simulink model "CochlearImplant_SIL"  (R2026b)
settings: Solver=FixedStepDiscrete  StopTime=5
PreLoadFcn:
  | addpath(fileparts(which('CochlearImplant_SIL')));
PostLoadFcn:
  | load speech_dft.mat
InitFcn:
  | dspcochlearfilterdesign;
  | source_type = 2;% 2 = Speech signal (1=Chirp)
  | filter_type = 1;% 1 = Cascade multirate FIR
  | noise_type  = 0;% 0 = no noise
  | denoise     = 0;% 0 = denoise off
StopFcn:
  | % Refresh OrigSignal/SynSignal in base from the latest run so the
  | % Play buttons never use stale data (robust to Single-simulation-output).
  | try
  |     if evalin('base','exist(''logsout'',''var'')')
  |         ls = evalin('base','logsout');
  |         if isa(ls,'Simulink.SimulationData.Dataset')
  |             if any(strcmp(ls.getElementNames,'InputSignal'))
  |                 assignin('base','OrigSignal', ls.get('InputSignal').Values.Data(:));
  |             end
  |             if any(strcmp(ls.getElementNames,'ReconSignal'))
  |                 assignin('base','SynSignal', ls.get('ReconSignal').Values.Data(:));
  |             end
  |         end
  |     end
  | catch ME
  |     warning('CochlearDemo:StopFcn','Could not refresh audio vars: %s', ME.message);
  | end
values from neighbouring files (symbols this model uses):
  cochleardemo_bpf = dsp.FIRFilter('Numerator', firls(32,[0 .22 .42 .54 .74 1], [0 0 1 1 0 0]))    [dspcochlearfilterdesign.m]
  cochleardemo_fir_hi = dsp.FIRFilter('Numerator', firls(32,[0 .62 .82 1], [0 0 1 1]))    [dspcochlearfilterdesign.m]
  cochleardemo_fir_lo = dsp.FIRFilter('Numerator', firls(32,[0 .62 .82 1], [1 1 0 0]))    [dspcochlearfilterdesign.m]
  cochleardemo_hpf = dsp.FIRFilter('Numerator', firls(32,[0 .54 .74 1], [0 0 1 1]))    [dspcochlearfilterdesign.m]
  cochleardemo_lpf = dsp.FIRFilter('Numerator', firls(32,[0 .22 .42  1], [1 1 0 0]))    [dspcochlearfilterdesign.m]
  fs = evalin('base', 'fs')    [plotFilterBankResponses.m]    (also in speech_dft.mat = 22050)
undefined symbols (not defined in the file or in its folder): cochleardemo_inputFilter, dfilt
libraries: dsparch4 x16, dspmlti4 x3, dspsrcs4 x1
settings Model: SILPILModeSetting=veronly  SimulationMode=software-in-the-loop (sil)  Creator=nkotwal  LastModifiedBy=jcchun
settings DataIOCC: ExternalInput=in  LoadExternalInput=on  ReturnWorkspaceOutputs=off  SignalLogging=off
settings OptimizationCC: DefaultParameterBehavior=Inlined  DifferentSizesBufferReuse=on  EfficientTunableParamExpr=on  EnhancedBackFolding=on  OptimizationCustomize=off  OptimizeBlockOrder=speed  PassReuseOutputArgsAs=Individual arguments  RemoveInternalMemoryZeroInit=on  RemoveRootLevelIOMemoryZeroInit=on
settings DebuggingCC: ParameterTunabilityLossMsg=error
settings HardwareCC: ProdHWDeviceType=AMD->x86-64 (Linux 64)
settings SFSimCC: MATLABDynamicMemAlloc=off
settings RTWCC: DataTypeReplacement=CDataTypesFixedWidth  Description=Embedded Coder  GenCodeOnly=on  GenerateCodeMetricsReport=on  GenerateReport=on  GenerateTraceInfo=on  IncludeHyperlinkInReport=on  SystemTargetFile=ert.tlc  TemplateMakefile=ert_default_tmf
settings CodeAppCC: ForceParamTrailComments=on  IgnoreCustomStorageClasses=off  InsertBlockDesc=on  OperatorAnnotations=on  SFDataObjDesc=on  SimulinkDataObjDesc=on
settings ERTTargetCC: CombineSignalStateStructs=on  GenerateSampleERTMain=on  MaxIdInt16=INT16_MAX  MaxIdInt32=INT32_MAX  MaxIdInt64=INT64_MAX  MaxIdInt8=INT8_MAX  MaxIdUint16=UINT16_MAX  MaxIdUint32=UINT32_MAX  MaxIdUint64=UINT64_MAX  MaxIdUint8=UINT8_MAX  MinIdInt16=INT16_MIN  MinIdInt32=INT32_MIN  MinIdInt64=INT64_MIN  MinIdInt8=INT8_MIN

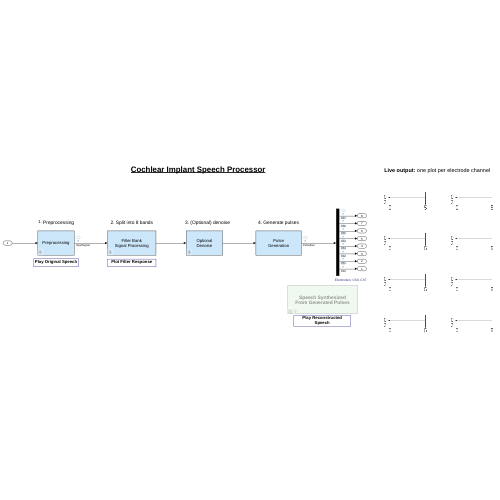
[thumbnail: Simulink's stored preview of the top-level diagram]
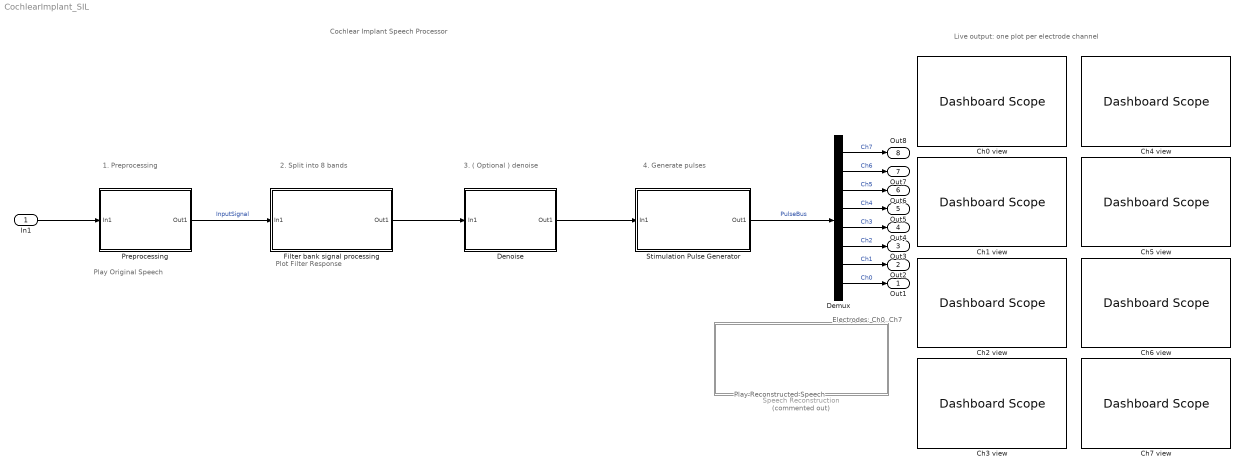
== system CochlearImplant_SIL ==
  note: Cochlear Implant Speech Processor
  note: 1. Preprocessing
  note: 2. Split into 8 bands
  note: 3. ( Optional ) denoise
  note: 4. Generate pulses
  note: Electrodes: Ch0..Ch7
  note: Live output: one plot per electrode channel
  note: Plot Filter Response
  note: Play Original Speech
  note: Play Reconstructed Speech
  In1 : Inport
  Ch0 view : DashboardScope  FontColor=[0.0, 0.0, 0.0]
  Ch1 view : DashboardScope  FontColor=[0.0, 0.0, 0.0]
  Ch2 view : DashboardScope  FontColor=[0.0, 0.0, 0.0]
  Ch3 view : DashboardScope  FontColor=[0.0, 0.0, 0.0]
  Ch4 view : DashboardScope  FontColor=[0.0, 0.0, 0.0]
  Ch5 view : DashboardScope  FontColor=[0.0, 0.0, 0.0]
  Ch6 view : DashboardScope  FontColor=[0.0, 0.0, 0.0]
  Ch7 view : DashboardScope  FontColor=[0.0, 0.0, 0.0]
  Demux : Demux  Outputs=8
  Denoise : Subsystem  mask{denoise=off}
      mask help: Apply soft thresholds to each filter bank output.
      mask Display: disp('Optional\nDenoise');
  Filter bank signal processing : Subsystem  mask(Filter bank signal processing){filter_type=Cascade multirate multi-stage FIR}
      mask prompts: filter_type "Filter bank:"
      mask help: Processes the input audio signal using a filter bank with eight subbands.
      mask TypeOptions filter_type: Cascade multirate multi-stage FIR | Parallel single-rate SOS IIR
      mask Display: disp('Filter Bank\nSignal Processing');
  Preprocessing : Subsystem  mask(Preprocessing){}
      mask Display: disp('Preprocessing');
  Speech Reconstruction : Subsystem  Commented=on  mask(Speech Synthesized From Generated Pulses){syn_mode=Play all channels at once}
      mask prompts: syn_mode "Synthesis mode:"
      mask help: Select whether to play all channels simultaneously or sequentially.
      mask TypeOptions syn_mode: Play all channels at once | Play channels sequentially
      mask Display: disp(sprintf('Speech Synthesized\nFrom Generated Pulses'));
  Stimulation Pulse Generator : Subsystem
      mask Display: disp('Pulse\nGeneration')
  Out1 : Outport
  Out2 : Outport  Port=2
  Out3 : Outport  Port=3
  Out4 : Outport  Port=4
  Out5 : Outport  Port=5
  Out6 : Outport  Port=6
  Out7 : Outport  Port=7
  Out8 : Outport  Port=8
  wires:
  Filter bank signal processing/1(Out1) -> Denoise/1(In1)
  Denoise/1(Out1) -> Stimulation Pulse Generator/1(In1)
  Stimulation Pulse Generator/1(Out1) -> Demux/1  "PulseBus"
  Preprocessing/1(Out1) -> Filter bank signal processing/1(In1)  "InputSignal"
  In1/1 -> Preprocessing/1(In1)
  Demux/8 -> Out1/1  "Ch0"
  Demux/7 -> Out2/1  "Ch1"
  Demux/6 -> Out3/1  "Ch2"
  Demux/5 -> Out4/1  "Ch3"
  Demux/4 -> Out5/1  "Ch4"
  Demux/3 -> Out6/1  "Ch5"
  Demux/2 -> Out7/1  "Ch6"
  Demux/1 -> Out8/1  "Ch7"

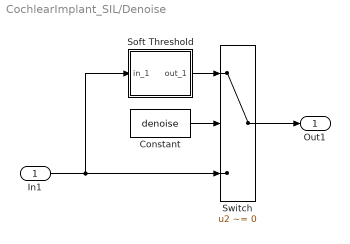
== system CochlearImplant_SIL/Denoise ==
  In1 : Inport
  Constant : Constant  Value=denoise
  Soft Threshold : Subsystem  mask(Soft Threshold){st=[0.5  0.3  0.2  0.2  0.2  0.2  0.2  0.2]}
      mask prompts: st "Vector of thresholds for each level:"
      mask help: Apply a soft threshold (deadzone transfer function) to each signal in the decomposition. First threshold applies to top-most filter bank output.
      mask init:
      | x=([-1 1 NaN 0 0 NaN -1 -.5 .5 1]+1)/2*.7+.15;
      | y=([0 0 NaN -1 1 NaN -1 0 0 1]+1)/2*.7+.05;
      mask Help: Vector of thresholds for each decomposition level.
      mask Display:
      | text(.1,.9,'Dead Zone')
      | plot(x,y)
  Switch : Switch  Criteria=u2 ~= 0  SaturateOnIntegerOverflow=off  InputSameDT=off
  Out1 : Outport  VectorParamsAs1DForOutWhenUnconnected=off
  wires:
  In1/1 -> Switch/3, Soft Threshold/1(in_1)
  Soft Threshold/1(out_1) -> Switch/1
  Switch/1 -> Out1/1
  Constant/1 -> Switch/2

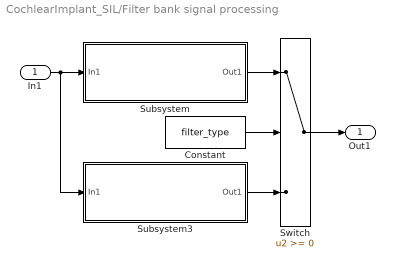
== system CochlearImplant_SIL/Filter bank signal processing ==
  In1 : Inport
  Constant : Constant  Value=filter_type
  Subsystem : Subsystem
      mask Display: disp('Cascade multirate multi-stage\nFIR filter bank');
  Subsystem3 : Subsystem
      mask Display: disp('Parallel single-rate\nSOS IIR filter bank');
  Switch : Switch  SaturateOnIntegerOverflow=off  InputSameDT=off
  Out1 : Outport  VectorParamsAs1DForOutWhenUnconnected=off
  wires:
  Switch/1 -> Out1/1
  In1/1 -> Subsystem3/1(In1), Subsystem/1(In1)
  Constant/1 -> Switch/2
  Subsystem3/1(Out1) -> Switch/3
  Subsystem/1(Out1) -> Switch/1

== system CochlearImplant_SIL/Preprocessing ==
  note: Input Preprocessing
  In1 : Inport
  Buffer : Buffer  N=8  ic=[0;0;0;0;0;3.0517578125e-05;-3.0517578125e-05;6.103515625e-05]
  DC Blocking Filter : DiscreteFilter  Numerator=cochleardemo_inputFilter.b  Denominator=cochleardemo_inputFilter.a  InputProcessing=Columns as channels (frame based)  FilterStructure=Direct form II transposed  a0EqualsOne=on  NumAccumDataTypeStr=Inherit: Same as product output  DenAccumDataTypeStr=Inherit: Same as product output
  stw : ToWorkspace  VariableName=OrigSignal  SampleTime=-1
      settings: Save2DSignal=2-D array (concatenate along first dimension)
  Out1 : Outport  VectorParamsAs1DForOutWhenUnconnected=off
  wires:
  DC Blocking Filter/1 -> Out1/1, stw/1
  Buffer/1 -> DC Blocking Filter/1
  In1/1 -> Buffer/1

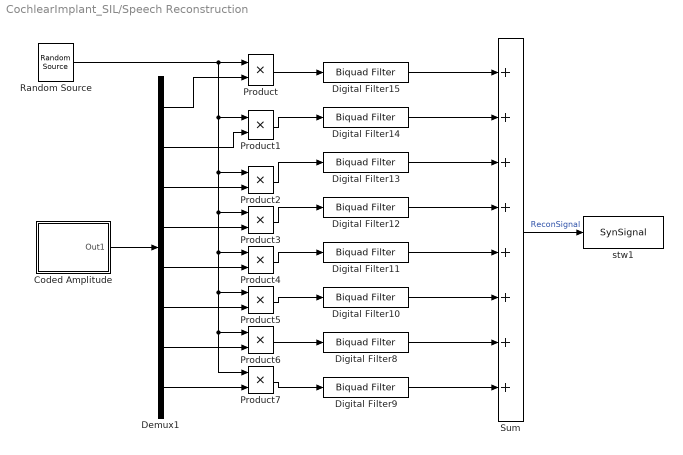
== system CochlearImplant_SIL/Speech Reconstruction ==
  Coded Amplitude : Subsystem
      mask Display: disp(['Speech' 10 'generated' 10 'pulses']);
  Demux1 : Demux  Outputs=8
  Digital Filter10 : dsparch4/Biquad Filter  FilterSource=Dialog parameters  CoeffSource=Specify via dialog  FilterObject=dfilt.df2tsos([1 0.3 0.4],[1 0.1 0.2])  IIRFiltStruct=Direct form II transposed  BiQuadCoeffs=cochleardemo_f2.sosMatrix  ScaleValues=cochleardemo_f2.ScaleValues  IC=0  ICnum=0  ICden=0  a0Flag=Error  optimizeScaleValues=on  ScaleValueMode=Specify via input port (g)  InputProcessing=Columns as channels (frame based)  roundingMode=Floor  overflowMode=off  scaleValueFracLength=14  denProdOutputFracLength=30  denAccumFracLength=30  secondMemoryFracLength=15
  Digital Filter11 : dsparch4/Biquad Filter  FilterSource=Dialog parameters  CoeffSource=Specify via dialog  FilterObject=dfilt.df2tsos([1 0.3 0.4],[1 0.1 0.2])  IIRFiltStruct=Direct form II transposed  BiQuadCoeffs=cochleardemo_f3.sosMatrix  ScaleValues=cochleardemo_f3.ScaleValues  IC=0  ICnum=0  ICden=0  a0Flag=Error  optimizeScaleValues=on  ScaleValueMode=Specify via input port (g)  InputProcessing=Columns as channels (frame based)  roundingMode=Floor  overflowMode=off  scaleValueFracLength=14  denProdOutputFracLength=30  denAccumFracLength=30  secondMemoryFracLength=15
  Digital Filter12 : dsparch4/Biquad Filter  FilterSource=Dialog parameters  CoeffSource=Specify via dialog  FilterObject=dfilt.df2tsos([1 0.3 0.4],[1 0.1 0.2])  IIRFiltStruct=Direct form II transposed  BiQuadCoeffs=cochleardemo_f4.sosMatrix  ScaleValues=cochleardemo_f4.ScaleValues  IC=0  ICnum=0  ICden=0  a0Flag=Error  optimizeScaleValues=on  ScaleValueMode=Specify via input port (g)  InputProcessing=Columns as channels (frame based)  roundingMode=Floor  overflowMode=off  scaleValueFracLength=14  denProdOutputFracLength=30  denAccumFracLength=30  secondMemoryFracLength=15
  Digital Filter13 : dsparch4/Biquad Filter  FilterSource=Dialog parameters  CoeffSource=Specify via dialog  FilterObject=dfilt.df2tsos([1 0.3 0.4],[1 0.1 0.2])  IIRFiltStruct=Direct form II transposed  BiQuadCoeffs=cochleardemo_f5.sosMatrix  ScaleValues=cochleardemo_f5.ScaleValues  IC=0  ICnum=0  ICden=0  a0Flag=Error  optimizeScaleValues=on  ScaleValueMode=Specify via input port (g)  InputProcessing=Columns as channels (frame based)  roundingMode=Floor  overflowMode=off  scaleValueFracLength=14  denProdOutputFracLength=30  denAccumFracLength=30  secondMemoryFracLength=15
  Digital Filter14 : dsparch4/Biquad Filter  FilterSource=Dialog parameters  CoeffSource=Specify via dialog  FilterObject=dfilt.df2tsos([1 0.3 0.4],[1 0.1 0.2])  IIRFiltStruct=Direct form II transposed  BiQuadCoeffs=cochleardemo_f6.sosMatrix  ScaleValues=cochleardemo_f6.ScaleValues  IC=0  ICnum=0  ICden=0  a0Flag=Error  optimizeScaleValues=on  ScaleValueMode=Specify via input port (g)  InputProcessing=Columns as channels (frame based)  roundingMode=Floor  overflowMode=off  scaleValueFracLength=14  denProdOutputFracLength=30  denAccumFracLength=30  secondMemoryFracLength=15
  Digital Filter15 : dsparch4/Biquad Filter  FilterSource=Dialog parameters  CoeffSource=Specify via dialog  FilterObject=dfilt.df2tsos([1 0.3 0.4],[1 0.1 0.2])  IIRFiltStruct=Direct form II transposed  BiQuadCoeffs=cochleardemo_f7.sosMatrix  ScaleValues=cochleardemo_f7.ScaleValues  IC=0  ICnum=0  ICden=0  a0Flag=Error  optimizeScaleValues=on  ScaleValueMode=Specify via input port (g)  InputProcessing=Columns as channels (frame based)  roundingMode=Floor  overflowMode=off  scaleValueFracLength=14  denProdOutputFracLength=30  denAccumFracLength=30  secondMemoryFracLength=15
  Digital Filter8 : dsparch4/Biquad Filter  FilterSource=Dialog parameters  CoeffSource=Specify via dialog  FilterObject=dfilt.df2tsos([1 0.3 0.4],[1 0.1 0.2])  IIRFiltStruct=Direct form II transposed  BiQuadCoeffs=cochleardemo_f1.sosMatrix  ScaleValues=cochleardemo_f1.ScaleValues  IC=0  ICnum=0  ICden=0  a0Flag=Error  optimizeScaleValues=on  ScaleValueMode=Specify via input port (g)  InputProcessing=Columns as channels (frame based)  roundingMode=Floor  overflowMode=off  scaleValueFracLength=14  denProdOutputFracLength=30  denAccumFracLength=30  secondMemoryFracLength=15
  Digital Filter9 : dsparch4/Biquad Filter  FilterSource=Dialog parameters  CoeffSource=Specify via dialog  FilterObject=dfilt.df2tsos([1 0.3 0.4],[1 0.1 0.2])  IIRFiltStruct=Direct form II transposed  BiQuadCoeffs=cochleardemo_f0.sosMatrix  ScaleValues=cochleardemo_f0.ScaleValues  IC=0  ICnum=0  ICden=0  a0Flag=Error  optimizeScaleValues=on  ScaleValueMode=Specify via input port (g)  InputProcessing=Columns as channels (frame based)  roundingMode=Floor  overflowMode=off  scaleValueFracLength=14  denProdOutputFracLength=30  denAccumFracLength=30  secondMemoryFracLength=15
  Product{,1..7} (8 alike) : Product  RndMeth=Zero
  Random Source : dspsrcs4/Random Source  SrcType=Uniform  MinVal=0  MaxVal=1  MeanVal=0  VarVal=1  RepMode=Specify seed  rawSeed=854301  IsInherit=off  SampTime=1/fs  SampFrame=8  OutComplex=Real  DataType=double  SimulateUsing=Interpreted execution
  Sum : Sum  Inputs=++++++++
  stw1 : ToWorkspace  VariableName=SynSignal  SampleTime=-1
      settings: Save2DSignal=2-D array (concatenate along first dimension)
  wires:
  Coded Amplitude/1(Out1) -> Demux1/1
  Digital Filter9/1 -> Sum/8
  Digital Filter8/1 -> Sum/7
  Digital Filter10/1 -> Sum/6
  Digital Filter11/1 -> Sum/5
  Digital Filter12/1 -> Sum/4
  Digital Filter13/1 -> Sum/3
  Digital Filter14/1 -> Sum/2
  Digital Filter15/1 -> Sum/1
  Demux1/8 -> Product7/2
  Demux1/7 -> Product6/2
  Demux1/6 -> Product5/2
  Demux1/5 -> Product4/2
  Demux1/4 -> Product3/2
  Demux1/3 -> Product2/2
  Demux1/2 -> Product1/2
  Demux1/1 -> Product/2
  Random Source/1 -> Product6/1, Product7/1, Product5/1, Product4/1, Product3/1, Product2/1, Product1/1, Product/1
  Sum/1 -> stw1/1  "ReconSignal"
  Product7/1 -> Digital Filter9/1
  Product6/1 -> Digital Filter8/1
  Product5/1 -> Digital Filter10/1
  Product4/1 -> Digital Filter11/1
  Product3/1 -> Digital Filter12/1
  Product2/1 -> Digital Filter13/1
  Product1/1 -> Digital Filter14/1
  Product/1 -> Digital Filter15/1

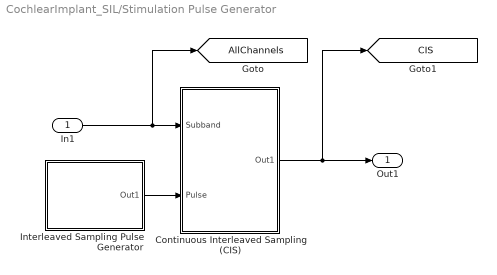
== system CochlearImplant_SIL/Stimulation Pulse Generator ==
  In1 : Inport
  Continuous Interleaved Sampling (CIS) : Subsystem
  Interleaved Sampling Pulse Generator : Subsystem
  Out1 : Outport  VectorParamsAs1DForOutWhenUnconnected=off
  tag scope: AllChannels=global, CIS=global
  wires:
  Continuous Interleaved Sampling (CIS)/1(Out1) -> [CIS], Out1/1
  In1/1 -> [AllChannels], Continuous Interleaved Sampling (CIS)/1(Subband)
  Interleaved Sampling Pulse Generator/1(Out1) -> Continuous Interleaved Sampling (CIS)/2(Pulse)

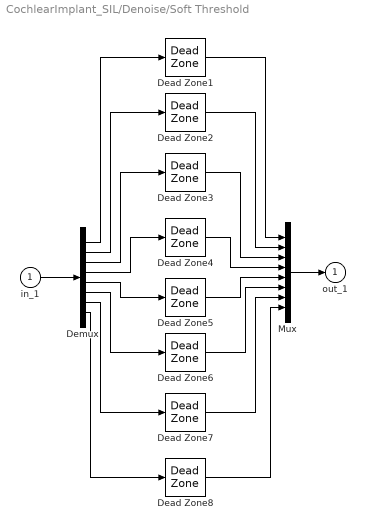
== system CochlearImplant_SIL/Denoise/Soft Threshold ==
  in_1 : Inport
  Dead Zone1 : DeadZone  LowerValue=-st(1)  UpperValue=st(1)  ZeroCross=off
  Dead Zone2 : DeadZone  LowerValue=-st(2)  UpperValue=st(2)  ZeroCross=off
  Dead Zone3 : DeadZone  LowerValue=-st(3)  UpperValue=st(3)  ZeroCross=off
  Dead Zone4 : DeadZone  LowerValue=-st(4)  UpperValue=st(4)  ZeroCross=off
  Dead Zone5 : DeadZone  LowerValue=-st(5)  UpperValue=st(5)  ZeroCross=off
  Dead Zone6 : DeadZone  LowerValue=-st(6)  UpperValue=st(6)  ZeroCross=off
  Dead Zone7 : DeadZone  LowerValue=-st(7)  UpperValue=st(7)  ZeroCross=off
  Dead Zone8 : DeadZone  LowerValue=-st(8)  UpperValue=st(8)  ZeroCross=off
  Demux : Demux  Outputs=8
  Mux : Mux  Inputs=8
  out_1 : Outport  VectorParamsAs1DForOutWhenUnconnected=off
  wires:
  in_1/1 -> Demux/1
  Demux/1 -> Dead Zone1/1
  Demux/2 -> Dead Zone2/1
  Demux/3 -> Dead Zone3/1
  Demux/4 -> Dead Zone4/1
  Demux/5 -> Dead Zone5/1
  Demux/6 -> Dead Zone6/1
  Demux/7 -> Dead Zone7/1
  Demux/8 -> Dead Zone8/1
  Mux/1 -> out_1/1
  Dead Zone1/1 -> Mux/1
  Dead Zone2/1 -> Mux/2
  Dead Zone3/1 -> Mux/3
  Dead Zone4/1 -> Mux/4
  Dead Zone5/1 -> Mux/5
  Dead Zone6/1 -> Mux/6
  Dead Zone7/1 -> Mux/7
  Dead Zone8/1 -> Mux/8

== system CochlearImplant_SIL/Filter bank signal processing/Subsystem ==
  In1 : Inport
  Cascade FIR Bank : Subsystem
  Rectifier : Subsystem
  Out1 : Outport  VectorParamsAs1DForOutWhenUnconnected=off
  wires:
  In1/1 -> Cascade FIR Bank/1(In1)
  Cascade FIR Bank/8(Out8) -> Rectifier/8(In8)
  Cascade FIR Bank/7(Out7) -> Rectifier/7(In7)
  Cascade FIR Bank/6(Out6) -> Rectifier/6(In6)
  Cascade FIR Bank/5(Out5) -> Rectifier/5(In5)
  Cascade FIR Bank/4(Out4) -> Rectifier/4(In4)
  Cascade FIR Bank/3(Out3) -> Rectifier/3(In3)
  Cascade FIR Bank/2(Out2) -> Rectifier/2(In2)
  Cascade FIR Bank/1(Out1) -> Rectifier/1(In1)
  Rectifier/1(Out1) -> Out1/1

== system CochlearImplant_SIL/Filter bank signal processing/Subsystem3 ==
  In1 : Inport
  IIR Filter Bank : Subsystem
  Rectifier : Subsystem
  Out1 : Outport  VectorParamsAs1DForOutWhenUnconnected=off
  wires:
  Rectifier/1(Out1) -> Out1/1
  IIR Filter Bank/1(Out1) -> Rectifier/1(In1)
  IIR Filter Bank/2(Out2) -> Rectifier/2(In2)
  IIR Filter Bank/3(Out3) -> Rectifier/3(In3)
  IIR Filter Bank/4(Out4) -> Rectifier/4(In4)
  IIR Filter Bank/5(Out5) -> Rectifier/5(In5)
  IIR Filter Bank/6(Out6) -> Rectifier/6(In6)
  IIR Filter Bank/7(Out7) -> Rectifier/7(In7)
  IIR Filter Bank/8(Out8) -> Rectifier/8(In8)
  In1/1 -> IIR Filter Bank/1(In1)

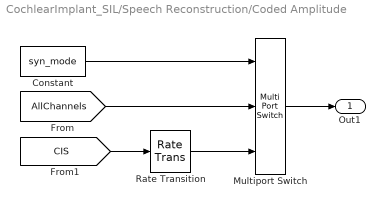
== system CochlearImplant_SIL/Speech Reconstruction/Coded Amplitude ==
  Constant : Constant  Value=syn_mode
  Multiport Switch : MultiPortSwitch  Inputs=2  SaturateOnIntegerOverflow=off  InputSameDT=off
  Rate Transition : RateTransition  OutPortSampleTime=8/fs
  Out1 : Outport  VectorParamsAs1DForOutWhenUnconnected=off
  wires:
  [CIS] -> Rate Transition/1
  Constant/1 -> Multiport Switch/1
  [AllChannels] -> Multiport Switch/2
  Rate Transition/1 -> Multiport Switch/3
  Multiport Switch/1 -> Out1/1

== system CochlearImplant_SIL/Stimulation Pulse Generator/Continuous Interleaved Sampling (CIS) ==
  Subband : Inport
  Pulse : Inport  Port=2
  Modulator : Product  RndMeth=Zero
  Rate Transition : RateTransition
  Out1 : Outport  VectorParamsAs1DForOutWhenUnconnected=off
  wires:
  Pulse/1 -> Modulator/2
  Subband/1 -> Rate Transition/1
  Modulator/1 -> Out1/1
  Rate Transition/1 -> Modulator/1

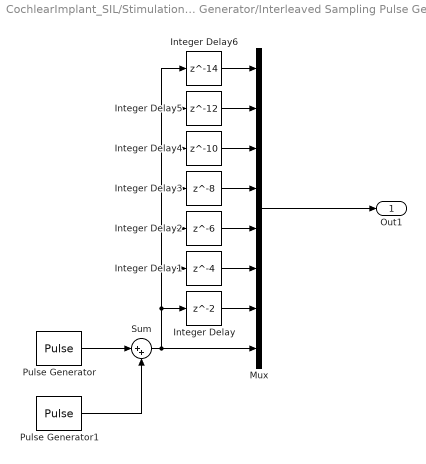
== system CochlearImplant_SIL/Stimulation Pulse Generator/Interleaved Sampling Pulse Generator ==
  Integer Delay : Delay
  Integer Delay1 : Delay  DelayLength=4
  Integer Delay2 : Delay  DelayLength=6
  Integer Delay3 : Delay  DelayLength=8
  Integer Delay4 : Delay  DelayLength=10
  Integer Delay5 : Delay  DelayLength=12
  Integer Delay6 : Delay  DelayLength=14
  Mux : Mux  Inputs=8
  Pulse Generator : DiscretePulseGenerator  Period=16  SampleTime=4/fs
  Pulse Generator1 : DiscretePulseGenerator  Amplitude=-1  Period=16  PhaseDelay=1  SampleTime=4/fs
  Sum : Sum  Inputs=|++
  Out1 : Outport  VectorParamsAs1DForOutWhenUnconnected=off
  wires:
  Sum/1 -> Integer Delay/1, Integer Delay1/1, Integer Delay2/1, Integer Delay3/1, Integer Delay4/1, Integer Delay5/1, Integer Delay6/1, Mux/8
  Integer Delay/1 -> Mux/7
  Integer Delay1/1 -> Mux/6
  Integer Delay2/1 -> Mux/5
  Integer Delay3/1 -> Mux/4
  Integer Delay4/1 -> Mux/3
  Integer Delay5/1 -> Mux/2
  Integer Delay6/1 -> Mux/1
  Pulse Generator/1 -> Sum/1
  Pulse Generator1/1 -> Sum/2
  Mux/1 -> Out1/1

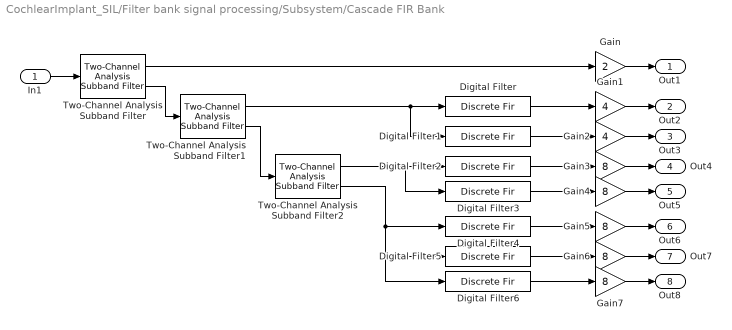
== system CochlearImplant_SIL/Filter bank signal processing/Subsystem/Cascade FIR Bank ==
  In1 : Inport
  Digital Filter : DiscreteFir  Coefficients=cochleardemo_fir_lo.Numerator  InputProcessing=Columns as channels (frame based)  AccumDataTypeStr=Inherit: Same as product output  OutDataTypeStr=Inherit: Same as accumulator
  Digital Filter1 : DiscreteFir  Coefficients=cochleardemo_fir_hi.Numerator  InputProcessing=Columns as channels (frame based)  AccumDataTypeStr=Inherit: Same as product output  OutDataTypeStr=Inherit: Same as accumulator
  Digital Filter2 : DiscreteFir  Coefficients=cochleardemo_fir_lo.Numerator  InputProcessing=Columns as channels (frame based)  AccumDataTypeStr=Inherit: Same as product output  OutDataTypeStr=Inherit: Same as accumulator
  Digital Filter3 : DiscreteFir  Coefficients=cochleardemo_fir_hi.Numerator  InputProcessing=Columns as channels (frame based)  AccumDataTypeStr=Inherit: Same as product output  OutDataTypeStr=Inherit: Same as accumulator
  Digital Filter4 : DiscreteFir  Coefficients=cochleardemo_hpf.Numerator  InputProcessing=Columns as channels (frame based)  AccumDataTypeStr=Inherit: Same as product output  OutDataTypeStr=Inherit: Same as accumulator
  Digital Filter5 : DiscreteFir  Coefficients=cochleardemo_bpf.Numerator  InputProcessing=Columns as channels (frame based)  AccumDataTypeStr=Inherit: Same as product output  OutDataTypeStr=Inherit: Same as accumulator
  Digital Filter6 : DiscreteFir  Coefficients=cochleardemo_lpf.Numerator  InputProcessing=Columns as channels (frame based)  AccumDataTypeStr=Inherit: Same as product output  OutDataTypeStr=Inherit: Same as accumulator
  Gain : Gain  Gain=2
  Gain1 : Gain  Gain=4
  Gain2 : Gain  Gain=4
  Gain{3..7} (5 alike) : Gain  Gain=8
  Two-Channel Analysis Subband Filter : dspmlti4/Two-Channel Analysis Subband Filter  lpf=cochleardemo_dec_lpf.Numerator  hpf=cochleardemo_dec_hpf.Numerator  InputProcessing=Columns as channels (frame based)  framing=Enforce single-rate processing  AllowArbitraryInputLength=off  roundingMode=Floor  overflowMode=off  firstCoeffDataTypeStr=Inherit: Same word length as input  firstCoeffMin=[]  firstCoeffMax=[]  firstCoeffLastDataTypeStr=Inherit: Same word length as input  outputDataTypeStr=Inherit: Same as accumulator  outputMin=[]  outputMax=[]  outputLastDataTypeStr=Inherit: Same as accumulator
  Two-Channel Analysis Subband Filter1 : dspmlti4/Two-Channel Analysis Subband Filter  lpf=cochleardemo_dec_lpf.Numerator  hpf=cochleardemo_dec_hpf.Numerator  InputProcessing=Columns as channels (frame based)  framing=Enforce single-rate processing  AllowArbitraryInputLength=off  roundingMode=Floor  overflowMode=off  firstCoeffDataTypeStr=Inherit: Same word length as input  firstCoeffMin=[]  firstCoeffMax=[]  firstCoeffLastDataTypeStr=Inherit: Same word length as input  outputDataTypeStr=Inherit: Same as accumulator  outputMin=[]  outputMax=[]  outputLastDataTypeStr=Inherit: Same as accumulator
  Two-Channel Analysis Subband Filter2 : dspmlti4/Two-Channel Analysis Subband Filter  lpf=cochleardemo_dec_lpf.Numerator  hpf=cochleardemo_dec_hpf.Numerator  InputProcessing=Columns as channels (frame based)  framing=Enforce single-rate processing  AllowArbitraryInputLength=off  roundingMode=Floor  overflowMode=off  firstCoeffDataTypeStr=Inherit: Same word length as input  firstCoeffMin=[]  firstCoeffMax=[]  firstCoeffLastDataTypeStr=Inherit: Same word length as input  outputDataTypeStr=Inherit: Same as accumulator  outputMin=[]  outputMax=[]  outputLastDataTypeStr=Inherit: Same as accumulator
  Out1 : Outport  VectorParamsAs1DForOutWhenUnconnected=off
  Out2 : Outport  Port=2  VectorParamsAs1DForOutWhenUnconnected=off
  Out3 : Outport  Port=3  VectorParamsAs1DForOutWhenUnconnected=off
  Out4 : Outport  Port=4  VectorParamsAs1DForOutWhenUnconnected=off
  Out5 : Outport  Port=5  VectorParamsAs1DForOutWhenUnconnected=off
  Out6 : Outport  Port=6  VectorParamsAs1DForOutWhenUnconnected=off
  Out7 : Outport  Port=7  VectorParamsAs1DForOutWhenUnconnected=off
  Out8 : Outport  Port=8  VectorParamsAs1DForOutWhenUnconnected=off
  wires:
  Two-Channel Analysis Subband Filter2/2 -> Digital Filter6/1, Digital Filter5/1, Digital Filter4/1
  Two-Channel Analysis Subband Filter2/1 -> Digital Filter3/1, Digital Filter2/1
  Two-Channel Analysis Subband Filter1/1 -> Digital Filter1/1, Digital Filter/1
  Two-Channel Analysis Subband Filter/1 -> Gain/1
  Gain7/1 -> Out8/1
  Gain6/1 -> Out7/1
  Gain5/1 -> Out6/1
  Gain4/1 -> Out5/1
  Gain3/1 -> Out4/1
  Gain2/1 -> Out3/1
  Gain1/1 -> Out2/1
  Gain/1 -> Out1/1
  In1/1 -> Two-Channel Analysis Subband Filter/1
  Two-Channel Analysis Subband Filter/2 -> Two-Channel Analysis Subband Filter1/1
  Digital Filter/1 -> Gain1/1
  Digital Filter1/1 -> Gain2/1
  Two-Channel Analysis Subband Filter1/2 -> Two-Channel Analysis Subband Filter2/1
  Digital Filter2/1 -> Gain3/1
  Digital Filter3/1 -> Gain4/1
  Digital Filter4/1 -> Gain5/1
  Digital Filter5/1 -> Gain6/1
  Digital Filter6/1 -> Gain7/1

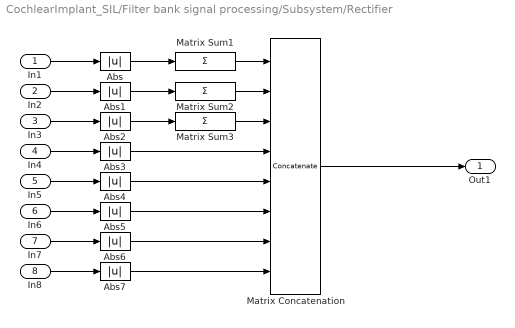
== system CochlearImplant_SIL/Filter bank signal processing/Subsystem/Rectifier ==
  In1 : Inport
  In2 : Inport  Port=2
  In3 : Inport  Port=3
  In4 : Inport  Port=4
  In5 : Inport  Port=5
  In6 : Inport  Port=6
  In7 : Inport  Port=7
  In8 : Inport  Port=8
  Abs{,1..7} (8 alike) : Abs  SaturateOnIntegerOverflow=off
  Matrix Concatenation : Concatenate  NumInputs=8  Mode=Multidimensional array
  Matrix Sum1 : Sum  Inputs=+  CollapseMode=Specified dimension  OutDataTypeStr=Inherit: Same as first input
  Matrix Sum2 : Sum  Inputs=+  CollapseMode=Specified dimension  OutDataTypeStr=Inherit: Same as first input
  Matrix Sum3 : Sum  Inputs=+  CollapseMode=Specified dimension  OutDataTypeStr=Inherit: Same as first input
  Out1 : Outport  VectorParamsAs1DForOutWhenUnconnected=off
  wires:
  Abs7/1 -> Matrix Concatenation/8
  Abs6/1 -> Matrix Concatenation/7
  Abs5/1 -> Matrix Concatenation/6
  Abs4/1 -> Matrix Concatenation/5
  Abs3/1 -> Matrix Concatenation/4
  Matrix Concatenation/1 -> Out1/1
  Matrix Sum3/1 -> Matrix Concatenation/3
  Matrix Sum2/1 -> Matrix Concatenation/2
  Matrix Sum1/1 -> Matrix Concatenation/1
  In8/1 -> Abs7/1
  In7/1 -> Abs6/1
  In6/1 -> Abs5/1
  In5/1 -> Abs4/1
  In4/1 -> Abs3/1
  In3/1 -> Abs2/1
  In2/1 -> Abs1/1
  In1/1 -> Abs/1
  Abs/1 -> Matrix Sum1/1
  Abs1/1 -> Matrix Sum2/1
  Abs2/1 -> Matrix Sum3/1

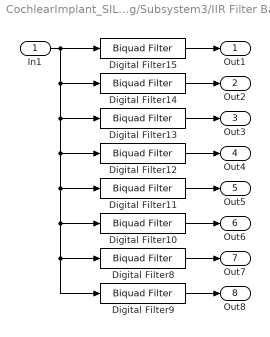
== system CochlearImplant_SIL/Filter bank signal processing/Subsystem3/IIR Filter Bank ==
  In1 : Inport
  Digital Filter10 : dsparch4/Biquad Filter  FilterSource=Dialog parameters  CoeffSource=Specify via dialog  FilterObject=dfilt.df2tsos([1 0.3 0.4],[1 0.1 0.2])  IIRFiltStruct=Direct form II transposed  BiQuadCoeffs=cochleardemo_f2.sosMatrix  ScaleValues=cochleardemo_f2.ScaleValues  IC=0  ICnum=0  ICden=0  a0Flag=Error  optimizeScaleValues=on  ScaleValueMode=Specify via input port (g)  InputProcessing=Columns as channels (frame based)  roundingMode=Floor  overflowMode=off  scaleValueFracLength=14  denProdOutputFracLength=30  denAccumFracLength=30  secondMemoryFracLength=15
  Digital Filter11 : dsparch4/Biquad Filter  FilterSource=Dialog parameters  CoeffSource=Specify via dialog  FilterObject=dfilt.df2tsos([1 0.3 0.4],[1 0.1 0.2])  IIRFiltStruct=Direct form II transposed  BiQuadCoeffs=cochleardemo_f3.sosMatrix  ScaleValues=cochleardemo_f3.ScaleValues  IC=0  ICnum=0  ICden=0  a0Flag=Error  optimizeScaleValues=on  ScaleValueMode=Specify via input port (g)  InputProcessing=Columns as channels (frame based)  roundingMode=Floor  overflowMode=off  scaleValueFracLength=14  denProdOutputFracLength=30  denAccumFracLength=30  secondMemoryFracLength=15
  Digital Filter12 : dsparch4/Biquad Filter  FilterSource=Dialog parameters  CoeffSource=Specify via dialog  FilterObject=dfilt.df2tsos([1 0.3 0.4],[1 0.1 0.2])  IIRFiltStruct=Direct form II transposed  BiQuadCoeffs=cochleardemo_f4.sosMatrix  ScaleValues=cochleardemo_f4.ScaleValues  IC=0  ICnum=0  ICden=0  a0Flag=Error  optimizeScaleValues=on  ScaleValueMode=Specify via input port (g)  InputProcessing=Columns as channels (frame based)  roundingMode=Floor  overflowMode=off  scaleValueFracLength=14  denProdOutputFracLength=30  denAccumFracLength=30  secondMemoryFracLength=15
  Digital Filter13 : dsparch4/Biquad Filter  FilterSource=Dialog parameters  CoeffSource=Specify via dialog  FilterObject=dfilt.df2tsos([1 0.3 0.4],[1 0.1 0.2])  IIRFiltStruct=Direct form II transposed  BiQuadCoeffs=cochleardemo_f5.sosMatrix  ScaleValues=cochleardemo_f5.ScaleValues  IC=0  ICnum=0  ICden=0  a0Flag=Error  optimizeScaleValues=on  ScaleValueMode=Specify via input port (g)  InputProcessing=Columns as channels (frame based)  roundingMode=Floor  overflowMode=off  scaleValueFracLength=14  denProdOutputFracLength=30  denAccumFracLength=30  secondMemoryFracLength=15
  Digital Filter14 : dsparch4/Biquad Filter  FilterSource=Dialog parameters  CoeffSource=Specify via dialog  FilterObject=dfilt.df2tsos([1 0.3 0.4],[1 0.1 0.2])  IIRFiltStruct=Direct form II transposed  BiQuadCoeffs=cochleardemo_f6.sosMatrix  ScaleValues=cochleardemo_f6.ScaleValues  IC=0  ICnum=0  ICden=0  a0Flag=Error  optimizeScaleValues=on  ScaleValueMode=Specify via input port (g)  InputProcessing=Columns as channels (frame based)  roundingMode=Floor  overflowMode=off  scaleValueFracLength=14  denProdOutputFracLength=30  denAccumFracLength=30  secondMemoryFracLength=15
  Digital Filter15 : dsparch4/Biquad Filter  FilterSource=Dialog parameters  CoeffSource=Specify via dialog  FilterObject=dfilt.df2tsos([1 0.3 0.4],[1 0.1 0.2])  IIRFiltStruct=Direct form II transposed  BiQuadCoeffs=cochleardemo_f7.sosMatrix  ScaleValues=cochleardemo_f7.ScaleValues  IC=0  ICnum=0  ICden=0  a0Flag=Error  optimizeScaleValues=on  ScaleValueMode=Specify via input port (g)  InputProcessing=Columns as channels (frame based)  roundingMode=Floor  overflowMode=off  scaleValueFracLength=14  denProdOutputFracLength=30  denAccumFracLength=30  secondMemoryFracLength=15
  Digital Filter8 : dsparch4/Biquad Filter  FilterSource=Dialog parameters  CoeffSource=Specify via dialog  FilterObject=dfilt.df2tsos([1 0.3 0.4],[1 0.1 0.2])  IIRFiltStruct=Direct form II transposed  BiQuadCoeffs=cochleardemo_f1.sosMatrix  ScaleValues=cochleardemo_f1.ScaleValues  IC=0  ICnum=0  ICden=0  a0Flag=Error  optimizeScaleValues=on  ScaleValueMode=Specify via input port (g)  InputProcessing=Columns as channels (frame based)  roundingMode=Floor  overflowMode=off  scaleValueFracLength=14  denProdOutputFracLength=30  denAccumFracLength=30  secondMemoryFracLength=15
  Digital Filter9 : dsparch4/Biquad Filter  FilterSource=Dialog parameters  CoeffSource=Specify via dialog  FilterObject=dfilt.df2tsos([1 0.3 0.4],[1 0.1 0.2])  IIRFiltStruct=Direct form II transposed  BiQuadCoeffs=cochleardemo_f0.sosMatrix  ScaleValues=cochleardemo_f0.ScaleValues  IC=0  ICnum=0  ICden=0  a0Flag=Error  optimizeScaleValues=on  ScaleValueMode=Specify via input port (g)  InputProcessing=Columns as channels (frame based)  roundingMode=Floor  overflowMode=off  scaleValueFracLength=14  denProdOutputFracLength=30  denAccumFracLength=30  secondMemoryFracLength=15
  Out1 : Outport  VectorParamsAs1DForOutWhenUnconnected=off
  Out2 : Outport  Port=2  VectorParamsAs1DForOutWhenUnconnected=off
  Out3 : Outport  Port=3  VectorParamsAs1DForOutWhenUnconnected=off
  Out4 : Outport  Port=4  VectorParamsAs1DForOutWhenUnconnected=off
  Out5 : Outport  Port=5  VectorParamsAs1DForOutWhenUnconnected=off
  Out6 : Outport  Port=6  VectorParamsAs1DForOutWhenUnconnected=off
  Out7 : Outport  Port=7  VectorParamsAs1DForOutWhenUnconnected=off
  Out8 : Outport  Port=8  VectorParamsAs1DForOutWhenUnconnected=off
  wires:
  In1/1 -> Digital Filter15/1, Digital Filter14/1, Digital Filter13/1, Digital Filter12/1, Digital Filter11/1, Digital Filter10/1, Digital Filter9/1, Digital Filter8/1
  Digital Filter15/1 -> Out1/1
  Digital Filter14/1 -> Out2/1
  Digital Filter13/1 -> Out3/1
  Digital Filter12/1 -> Out4/1
  Digital Filter11/1 -> Out5/1
  Digital Filter10/1 -> Out6/1
  Digital Filter8/1 -> Out7/1
  Digital Filter9/1 -> Out8/1

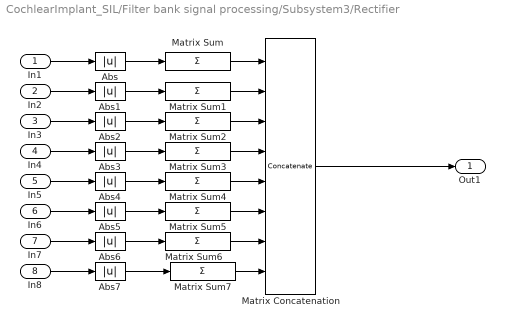
== system CochlearImplant_SIL/Filter bank signal processing/Subsystem3/Rectifier ==
  In1 : Inport
  In2 : Inport  Port=2
  In3 : Inport  Port=3
  In4 : Inport  Port=4
  In5 : Inport  Port=5
  In6 : Inport  Port=6
  In7 : Inport  Port=7
  In8 : Inport  Port=8
  Abs{,1..7} (8 alike) : Abs  SaturateOnIntegerOverflow=off
  Matrix Concatenation : Concatenate  NumInputs=8  Mode=Multidimensional array
  Matrix Sum{,1..7} (8 alike) : Sum  Inputs=+  CollapseMode=Specified dimension  OutDataTypeStr=Inherit: Same as first input
  Out1 : Outport  VectorParamsAs1DForOutWhenUnconnected=off
  wires:
  Matrix Concatenation/1 -> Out1/1
  Abs7/1 -> Matrix Sum7/1
  Abs6/1 -> Matrix Sum6/1
  Abs5/1 -> Matrix Sum5/1
  Abs4/1 -> Matrix Sum4/1
  Abs3/1 -> Matrix Sum3/1
  Matrix Sum2/1 -> Matrix Concatenation/3
  Matrix Sum1/1 -> Matrix Concatenation/2
  Matrix Sum/1 -> Matrix Concatenation/1
  In8/1 -> Abs7/1
  In7/1 -> Abs6/1
  In6/1 -> Abs5/1
  In5/1 -> Abs4/1
  In4/1 -> Abs3/1
  In3/1 -> Abs2/1
  In2/1 -> Abs1/1
  In1/1 -> Abs/1
  Abs/1 -> Matrix Sum/1
  Abs1/1 -> Matrix Sum1/1
  Abs2/1 -> Matrix Sum2/1
  Matrix Sum3/1 -> Matrix Concatenation/4
  Matrix Sum4/1 -> Matrix Concatenation/5
  Matrix Sum5/1 -> Matrix Concatenation/6
  Matrix Sum6/1 -> Matrix Concatenation/7
  Matrix Sum7/1 -> Matrix Concatenation/8
